simulink model "innerLoopForNav"  (R2024b)
settings: Solver=ode4  StartTime=0.0  StopTime=60  FixedStep=0.02  RelTol=1e-3
undefined symbols (not defined in the file): euler_0, V_0
libraries: simulink x7
settings Model: Creator=yuanjiayi  LastModifiedBy=yuanjiayi

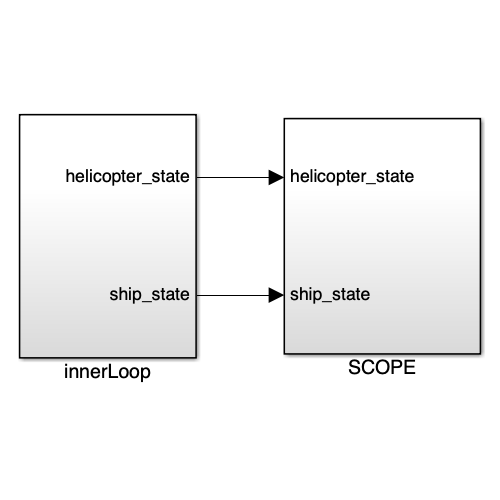
[thumbnail: Simulink's stored preview of the top-level diagram]
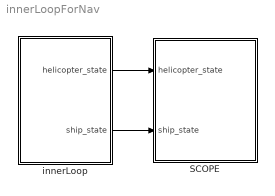
== system innerLoopForNav ==
  SCOPE : Subsystem
  innerLoop : Subsystem
  wires:
  innerLoop/1(helicopter_state) -> SCOPE/1(helicopter_state)
  innerLoop/2(ship_state) -> SCOPE/2(ship_state)

== system innerLoopForNav/SCOPE ==
  helicopter_state : Inport
  ship_state : Inport  Port=2
  Demux1 : Demux  Outputs=12
  Demux2 : Demux  Outputs=12
  Scope : Scope  NumInputPorts=12
  Scope1 : Scope  NumInputPorts=12
  wires:
  Demux2/6 -> Scope1/6  "w"
  Demux2/2 -> Scope1/2  "y"
  helicopter_state/1 -> Demux1/1
  Demux1/1 -> Scope/1  "x"
  Demux1/3 -> Scope/3  "z"
  Demux1/12 -> Scope/12  "r"
  Demux2/9 -> Scope1/9  "psi"
  Demux1/9 -> Scope/9  "psi"
  Demux2/5 -> Scope1/5  "v"
  Demux1/7 -> Scope/7  "phi"
  Demux1/11 -> Scope/11  "q"
  Demux2/4 -> Scope1/4  "u"
  Demux1/2 -> Scope/2  "y"
  Demux1/8 -> Scope/8  "theta"
  Demux1/5 -> Scope/5  "v"
  Demux2/11 -> Scope1/11  "q"
  Demux2/12 -> Scope1/12  "r"
  ship_state/1 -> Demux2/1
  Demux2/3 -> Scope1/3  "z"
  Demux1/10 -> Scope/10  "p"
  Demux2/10 -> Scope1/10  "p"
  Demux2/1 -> Scope1/1  "x"
  Demux2/7 -> Scope1/7  "phi"
  Demux1/4 -> Scope/4  "u"
  Demux2/8 -> Scope1/8  "theta"
  Demux1/6 -> Scope/6  "w"

== system innerLoopForNav/innerLoop ==
  HELI_CONT : Subsystem
  LAND_CMD : Subsystem
  Mux : Mux  Inputs=2
  Plus : Sum
  mps2knots : Gain  Gain=[1/0.514444;1/0.514444;1/0.514444;1;1;1;1;1;1]
  mps2knots1 : Gain  Gain=[1;1;1;1/0.514444;1/0.514444;1/0.514444;1;1;1;1;1;1]
  relistedStates : Selector  InputPortWidth=9  IndexOptions=Index vector (dialog)  Indices=[1 5 2 8 4 9 6 3 7]  OutputSizes=1
  trim_9states : Constant  Value=[V_0; euler_0;zeros(3,1)]
  helicopter_state : Outport
  ship_state : Outport  Port=2
  wires:
  LAND_CMD/1(ref /knots) -> HELI_CONT/1(ref_ned)  "ref_ned / knots"
  LAND_CMD/3(xyz_heli) -> Mux/1
  Mux/1 -> helicopter_state/1
  HELI_CONT/1(V_ned) -> LAND_CMD/1(V_ned / knots)  "V_ned / knots"
  HELI_CONT/2(9states_heli) -> relistedStates/1
  LAND_CMD/2(ship_state) -> mps2knots1/1
  relistedStates/1 -> Plus/1
  Plus/1 -> mps2knots/1
  trim_9states/1 -> Plus/2
  mps2knots/1 -> Mux/2
  mps2knots1/1 -> ship_state/1

== system innerLoopForNav/innerLoop/HELI_CONT ==
  ref_ned : Inport
  SCOPE : Subsystem
  Some methods : Subsystem  Commented=on
  UWV_CONT : Subsystem
  nedToUwv : Subsystem
  V_ned : Outport
  9states_heli : Outport  Port=2
  wires:
  ref_ned/1 -> [ref_ned], nedToUwv/1(In1)
  UWV_CONT/2(euler) -> [euler]
  UWV_CONT/1(V_ned) -> V_ned/1, [V_ned]
  [euler] -> nedToUwv/2(In2)  "eluer / rad"
  nedToUwv/1(ref) -> UWV_CONT/1(ref)  "ref_u,w,v"
  [ref_ned] -> SCOPE/1(ref_ned)
  [V_ned] -> SCOPE/2(V_ned)
  UWV_CONT/3(9states_heli) -> 9states_heli/1

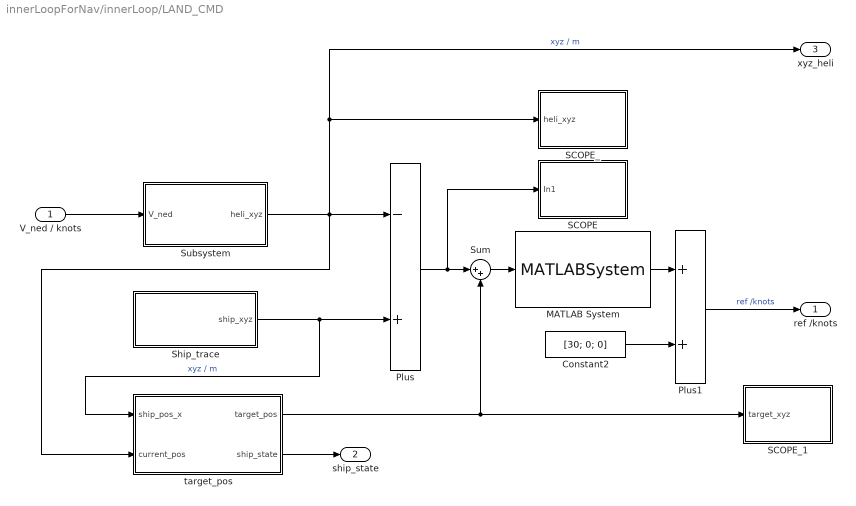
== system innerLoopForNav/innerLoop/LAND_CMD ==
  V_ned / knots : Inport
  Constant2 : Constant  Value=[30; 0; 0]
  MATLAB System : MATLABSystem  System=uvw_Gen  maxDeltaVel_n=1.5  maxDeltaVel_e=0.5  maxDeltaVel_d=1.5  SimulateUsing=Code generation
      mask Type: uvw_Gen
      mask Display:
      | disp('uvw_Gen');
      | port_label('input',1,'Delta_r');
      | port_label('output',1,'Delta_v');
  Plus : Sum  Inputs=-+
  Plus1 : Sum
  "SCOPE " : Subsystem
  SCOPE_ : Subsystem
  SCOPE_1 : Subsystem
  Ship_trace : Subsystem
  Subsystem : Subsystem
  Sum : Sum  Inputs=|++
  target_pos : Subsystem
  ref /knots : Outport
  ship_state : Outport  Port=2
  xyz_heli : Outport  Port=3
  wires:
  Constant2/1 -> Plus1/2
  Plus1/1 -> ref /knots/1  "ref /knots"
  V_ned / knots/1 -> Subsystem/1(V_ned)
  MATLAB System/1 -> Plus1/1
  Subsystem/1(heli_xyz) -> Plus/1, SCOPE_/1(heli_xyz), xyz_heli/1, target_pos/2(current_pos)  "xyz / m"
  Plus/1 -> "SCOPE "/1(In1), Sum/1
  Ship_trace/1(ship_xyz) -> Plus/2, target_pos/1(ship_pos_x)  "xyz / m"
  target_pos/1(target_pos) -> Sum/2, SCOPE_1/1(target_xyz)
  target_pos/2(ship_state) -> ship_state/1
  Sum/1 -> MATLAB System/1

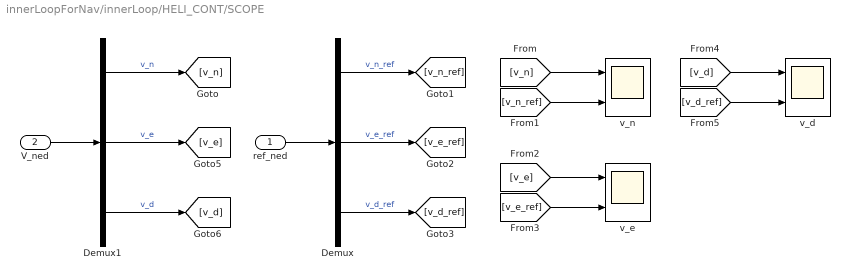
== system innerLoopForNav/innerLoop/HELI_CONT/SCOPE ==
  ref_ned : Inport
  V_ned : Inport  Port=2
  Demux : Demux  Outputs=3
  Demux1 : Demux  Outputs=3
  v_d : Scope  NumInputPorts=2
  v_e : Scope  NumInputPorts=2
  v_n : Scope  NumInputPorts=2
  wires:
  ref_ned/1 -> Demux/1
  V_ned/1 -> Demux1/1
  Demux1/1 -> [v_n]  "v_n"
  Demux/1 -> [v_n_ref]  "v_n_ref"
  [v_n] -> v_n/1
  [v_n_ref] -> v_n/2
  Demux/2 -> [v_e_ref]  "v_e_ref"
  Demux/3 -> [v_d_ref]  "v_d_ref"
  Demux1/2 -> [v_e]  "v_e"
  Demux1/3 -> [v_d]  "v_d"
  [v_e] -> v_e/1
  [v_e_ref] -> v_e/2
  [v_d] -> v_d/1
  [v_d_ref] -> v_d/2

== system innerLoopForNav/innerLoop/HELI_CONT/Some methods ==
  NDI_ : Subsystem  Commented=on
  PID_ : Subsystem  Commented=on
  reference signal : Subsystem  Commented=on

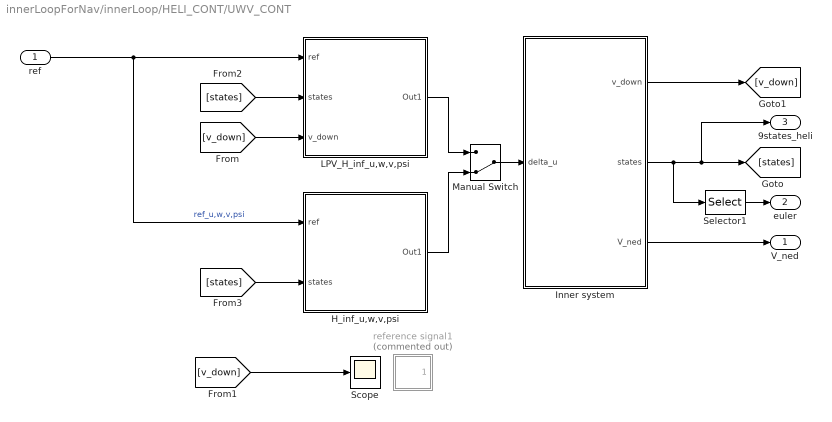
== system innerLoopForNav/innerLoop/HELI_CONT/UWV_CONT ==
  ref : Inport
  H_inf_u,w,v,psi : Subsystem
  Inner system : Subsystem
  LPV_H_inf_u,w,v,psi : Subsystem
  Manual Switch : ManualSwitch  CurrentSetting=0
  Scope : Scope
  Selector1 : Selector  InputPortWidth=9  IndexOptions=Index vector (dialog)  Indices=[8 4 9]  OutputSizes=1
  reference signal1 : Subsystem  Commented=on
  V_ned : Outport
  euler : Outport  Port=2
  9states_heli : Outport  Port=3
  wires:
  Inner system/1(v_down) -> [v_down]
  Inner system/2(states) -> 9states_heli/1, [states], Selector1/1
  Inner system/3(V_ned) -> V_ned/1
  ref/1 -> H_inf_u,w,v,psi/1(ref), LPV_H_inf_u,w,v,psi/1(ref)  "ref_u,w,v,psi"
  [states] -> LPV_H_inf_u,w,v,psi/2(states)
  [v_down] -> LPV_H_inf_u,w,v,psi/3(v_down)
  [v_down] -> Scope/1
  Selector1/1 -> euler/1
  LPV_H_inf_u,w,v,psi/1(Out1) -> Manual Switch/1
  Manual Switch/1 -> Inner system/1(delta_u)
  H_inf_u,w,v,psi/1(Out1) -> Manual Switch/2
  [states] -> H_inf_u,w,v,psi/2(states)

== system innerLoopForNav/innerLoop/HELI_CONT/nedToUwv ==
  In1 : Inport
  In2 : Inport  Port=2
  Constant : Constant  Value=0
  Constant2 : Constant  Value=[V_0]
  Demux2 : Demux  Outputs=3
  Gain : Gain  Gain=0.514444
  MATLAB System : MATLABSystem  System=nedVelToBody  SimulateUsing=Code generation
      mask Type: nedVelToBody
      mask Display:
      | disp('nedVelToBody');
      | port_label('input',1,'V_ned');
      | port_label('input',2,'Euler');
      | port_label('output',1,'V_body');
  Mux : Mux  Inputs=2
  Plus : Sum  Inputs=+-
  Scope3 : Scope  NumInputPorts=3
  Selector : Selector  InputPortWidth=3  IndexOptions=Index vector (dialog)  Indices=[1 3 2]  OutputSizes=1
  filter_phi,theta,psi : Subsystem
  filter_u,w,v,psi : Subsystem  Commented=on
  ref : Outport
  wires:
  filter_phi,theta,psi/1(Out1) -> MATLAB System/2
  Demux2/2 -> Scope3/2  "v"
  Demux2/3 -> Scope3/3  "w"
  In2/1 -> filter_phi,theta,psi/1(In1)
  MATLAB System/1 -> Plus/1, Demux2/1  "V_body_ref"
  Constant/1 -> Mux/2
  In1/1 -> Gain/1
  Demux2/1 -> Scope3/1  "u"
  Plus/1 -> Selector/1
  Constant2/1 -> Plus/2  "V_body_trim"
  Selector/1 -> Mux/1
  Gain/1 -> MATLAB System/1
  Mux/1 -> ref/1

== system innerLoopForNav/innerLoop/LAND_CMD/SCOPE  ==
  In1 : Inport
  Demux : Demux  Outputs=3
  Scope : Scope  NumInputPorts=3
  wires:
  Demux/3 -> Scope/3  "delta_z"
  In1/1 -> Demux/1
  Demux/2 -> Scope/2  "delta_y"
  Demux/1 -> Scope/1  "delta_x"

== system innerLoopForNav/innerLoop/LAND_CMD/SCOPE_ ==
  heli_xyz : Inport
  Demux : Demux  Outputs=3
  Gain : Gain  Gain=-1
  MATLAB Function : MATLAB Function  TreatAsAtomicUnit=on
  Scope : Scope  NumInputPorts=3
  Stop Simulation : Stop
  To Workspace : ToWorkspace  VariableName=heli_trace  SampleTime=-1
  wires:
  Demux/3 -> Gain/1  "z"
  heli_xyz/1 -> To Workspace/1, Demux/1
  Demux/2 -> Scope/2  "y"
  Demux/1 -> Scope/1  "x"
  Gain/1 -> MATLAB Function/1(z), Scope/3  "z"
  MATLAB Function/1(shallStop) -> Stop Simulation/1

== system innerLoopForNav/innerLoop/LAND_CMD/SCOPE_1 ==
  target_xyz : Inport
  Demux : Demux  Outputs=3
  Gain : Gain  Gain=-1
  Scope : Scope  NumInputPorts=3
  wires:
  Demux/3 -> Gain/1  "z"
  target_xyz/1 -> Demux/1
  Demux/2 -> Scope/2  "y"
  Demux/1 -> Scope/1  "x"
  Gain/1 -> Scope/3

== system innerLoopForNav/innerLoop/LAND_CMD/Ship_trace ==
  Constant2 : Constant  Value=[30; 0; 0]
  Gain1 : Gain  Gain=0.514444
  Integrator1 : Integrator  InitialCondition=[95;0;0]
  ship_xyz : Outport
  wires:
  Gain1/1 -> Integrator1/1
  Integrator1/1 -> ship_xyz/1
  Constant2/1 -> Gain1/1

== system innerLoopForNav/innerLoop/LAND_CMD/Subsystem ==
  V_ned : Inport
  Gain : Gain  Gain=0.514444
  Integrator : Integrator  InitialCondition=[0;0;-50]
  heli_xyz : Outport
  wires:
  Integrator/1 -> heli_xyz/1
  V_ned/1 -> Gain/1
  Gain/1 -> Integrator/1

== system innerLoopForNav/innerLoop/LAND_CMD/target_pos ==
  ship_pos_x : Inport
  current_pos : Inport  Port=2
  Chart : Stateflow chart  TreatAsAtomicUnit=on
  PredictModel : Subsystem
  Scope : Scope
  Selector : Selector  InputPortWidth=3  IndexOptions=Index vector (dialog)  Indices=[3]  OutputSizes=1
  Selector1 : Selector  InputPortWidth=3  IndexOptions=Index vector (dialog)  Indices=[1]  OutputSizes=1
  Selector2 : Selector  InputPortWidth=3  IndexOptions=Index vector (dialog)  Indices=[1]  OutputSizes=1
  Ship_motion : Subsystem
  To Workspace : ToWorkspace  VariableName=process_state  SampleTime=-1
  vel_cmd : Constant  Value=[30 ;0;0]
  target_pos : Outport
  ship_state : Outport  Port=2
  wires:
  vel_cmd/1 -> Ship_motion/1(In2), PredictModel/1(In2)
  current_pos/1 -> Selector/1, Selector1/1
  Selector/1 -> Chart/2(z)
  PredictModel/1(EI) -> Chart/1(EI)
  Chart/1(target_pos) -> target_pos/1
  Chart/2(state) -> To Workspace/1, Scope/1
  Ship_motion/1(ship_state) -> ship_state/1
  Selector1/1 -> Chart/3(x)
  ship_pos_x/1 -> Selector2/1
  Selector2/1 -> Chart/4(ship_pos_x)

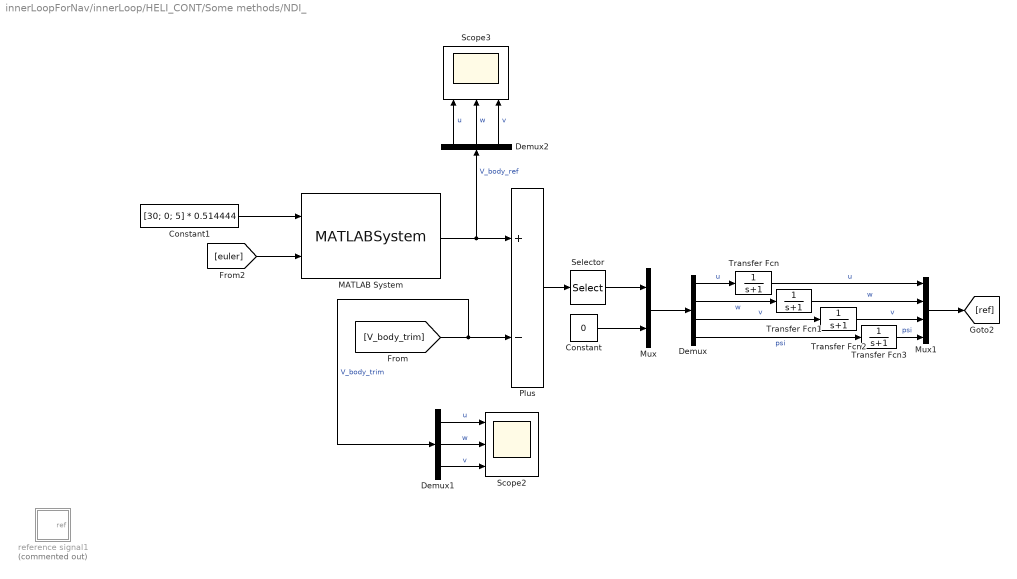
== system innerLoopForNav/innerLoop/HELI_CONT/Some methods/NDI_ ==
  Constant : Constant  Value=0
  Constant1 : Constant  Value=[30; 0; 5] * 0.514444
  Demux : Demux
  Demux1 : Demux  Outputs=3
  Demux2 : Demux  Outputs=3
  MATLAB System : MATLABSystem  System=nedVelToBody  SimulateUsing=Code generation
      mask Type: nedVelToBody
      mask Display:
      | disp('nedVelToBody');
      | port_label('input',1,'V_ned');
      | port_label('input',2,'Euler');
      | port_label('output',1,'V_body');
  Mux : Mux  Inputs=2
  Mux1 : Mux
  Plus : Sum  Inputs=+-
  Scope2 : Scope  NumInputPorts=3
  Scope3 : Scope  NumInputPorts=3
  Selector : Selector  InputPortWidth=3  IndexOptions=Index vector (dialog)  Indices=[1 3 2]  OutputSizes=1
  Transfer Fcn{,1..3} (4 alike) : TransferFcn  Denominator=[1 1]
  reference signal1 : Subsystem  Commented=on
  wires:
  Demux/3 -> Transfer Fcn2/1  "v"
  Demux2/2 -> Scope3/2  "w"
  Demux1/1 -> Scope2/1  "u"
  Mux/1 -> Demux/1
  MATLAB System/1 -> Plus/1, Demux2/1  "V_body_ref"
  Transfer Fcn3/1 -> Mux1/4  "psi"
  Demux2/3 -> Scope3/3  "v"
  Demux1/2 -> Scope2/2  "w"
  Constant1/1 -> MATLAB System/1
  Demux/1 -> Transfer Fcn/1  "u"
  Plus/1 -> Selector/1
  Mux1/1 -> [ref]
  Transfer Fcn1/1 -> Mux1/2  "w"
  Selector/1 -> Mux/1
  [euler] -> MATLAB System/2
  Demux/2 -> Transfer Fcn1/1  "w"
  Transfer Fcn/1 -> Mux1/1  "u"
  [V_body_trim] -> Demux1/1, Plus/2  "V_body_trim"
  Demux/4 -> Transfer Fcn3/1  "psi"
  Transfer Fcn2/1 -> Mux1/3  "v"
  Demux2/1 -> Scope3/1  "u"
  Demux1/3 -> Scope2/3  "v"
  Constant/1 -> Mux/2

== system innerLoopForNav/innerLoop/HELI_CONT/Some methods/PID_ ==
  Gain : Gain  Gain=0.514444
  Mux : Mux  Inputs=3
  Mux1 : Mux  Inputs=2
  Plus : Sum  Inputs=+-
  Scope1 : Scope
  filter & selector : Subsystem
  psi_ref : Constant  Value=0
  v_d_ref / knots : Constant  Value=5.0
  v_e_ref / knots : Constant  Value=0
  v_n_ref / knots : Constant  Value=30
  Out1 : Outport
  wires:
  Mux1/1 -> Out1/1
  v_d_ref / knots/1 -> Mux/3
  psi_ref/1 -> Mux1/2
  filter & selector/1(Out1) -> Scope1/1, Gain/1
  Gain/1 -> Mux1/1
  [ned] -> Plus/2
  Mux/1 -> Plus/1
  v_n_ref / knots/1 -> Mux/1
  Plus/1 -> filter & selector/1(In1)
  v_e_ref / knots/1 -> Mux/2

== system innerLoopForNav/innerLoop/HELI_CONT/Some methods/reference signal ==
  Constant : Constant  Value=0.5
  Mux : Mux
  Sine Wave : Sin  Amplitude=0.0  Frequency=0.2  SampleTime=0
  Sine Wave2 : Sin  Amplitude=0.0  Frequency=0.15  Phase=pi / 4  SampleTime=0
  Sine Wave3 : Sin  Amplitude=0.0  Frequency=0.15  Phase=pi / 4  SampleTime=0
  Out1 : Outport
  wires:
  Sine Wave/1 -> Mux/1  "ref_delta_u"
  Mux/1 -> Out1/1
  Constant/1 -> Mux/2  "ref_delta_w"
  Sine Wave2/1 -> Mux/3  "ref_delta_v"
  Sine Wave3/1 -> Mux/4  "ref_delta_psi"

== system innerLoopForNav/innerLoop/HELI_CONT/UWV_CONT/H_inf_u,w,v,psi ==
  ref : Inport
  states : Inport  Port=2
  MATLAB System : MATLABSystem  System=H_inf  PlantA=A_0  PlantB=B_0  ControlledStateIndices=[ 1, 2, 5, 9]  SampleTime=0.02  DKIterations=10  SelectedIteration=6  FrequencyGrid=logspace( -3, 3, 300 )  DiscretizationMethod=tustin  PerformanceA=0.005  PerformanceM=2  PerformanceBandwidth=1  UncertaintyZero=0.2  UncertaintyDenS=0.5  UncertaintyDen0=1  EnableInputSaturation=false  InputLowerLimit=-0.01 * ones( 4, 1 )  InputUpperLimit=0.01 * ones( 4, 1 )  SimulateUsing=Interpreted execution
      mask Type: H_inf
      mask Display:
      | disp('H_inf');
      | port_label('input',1,'r');
      | port_label('input',2,'y');
      | port_label('output',1,'delta');
  SCOPE : Subsystem
  Selector2 : Selector  InputPortWidth=9  IndexOptions=Index vector (dialog)  Indices=[1 2 5 9]  OutputSizes=1
  Out1 : Outport
  wires:
  states/1 -> Selector2/1
  Selector2/1 -> MATLAB System/2, SCOPE/2(y)  "u,w,v,psi"
  MATLAB System/1 -> Out1/1
  ref/1 -> MATLAB System/1, SCOPE/1(ref)

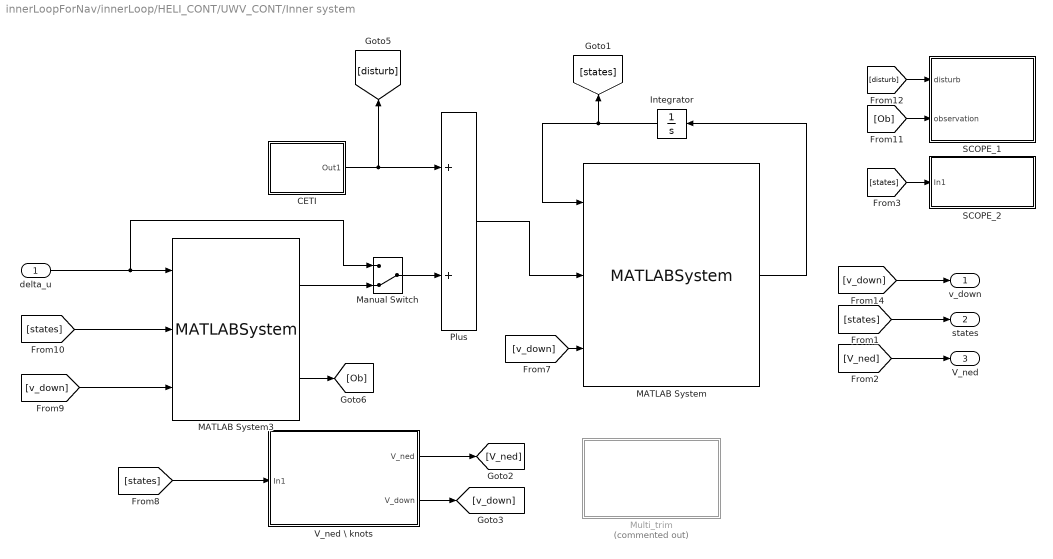
== system innerLoopForNav/innerLoop/HELI_CONT/UWV_CONT/Inner system ==
  delta_u : Inport
  CETI : Subsystem
  Integrator : Integrator  InitialCondition=[0.0;0.0;0.0;0.0;0.0;0.0;0.0;0.0;0.0]
  MATLAB System : MATLABSystem  System=multi_lin_sys  A_10=A_10  B_10=B_10  A_5=A_5  B_5=B_5  A_0=A_0  B_0=B_0  ClampSchedulingVariable=true  SimulateUsing=Interpreted execution
      mask Type: multi_lin_sys
      mask Display:
      | disp('multi_lin_sys');
      | port_label('input',1,'x');
      | port_label('input',2,'delta');
      | port_label('input',3,'v_down');
      | port_label('output',1,'x_dot');
  MATLAB System3 : MATLABSystem  System=LPV_NDO  A_10=A_10  B_10=B_10  A_5=A_5  B_5=B_5  A_0=A_0  B_0=B_0  SampleTime=0.02  ObserverBandwidth=50  ObserverGain_10=[]  ObserverGain_5=[]  ObserverGain_0=[]  DisturbanceFilterBandwidth=0  EnableDisturbanceLimit=true  DisturbanceLowerLimit=[ -0.05; -0.05; -0.05; -0.05 ]  DisturbanceUpperLimit=[ 0.05; 0.05; 0.05; 0.05 ]  EnableInputSaturation=false  InputLowerLimit=[ -inf; -inf; -inf; -inf ]  InputUpperLimit=[ inf; inf; inf; inf ]  ClampSchedulingVariable=true  SimulateUsing=Code generation
      mask Type: LPV_NDO
      mask Display:
      | disp('LPV_NDO');
      | port_label('input',1,'u0');
      | port_label('input',2,'x');
      | port_label('input',3,'v_down');
      | port_label('output',1,'u_comp');
      | port_label('output',2,'d_hat');
  Manual Switch : ManualSwitch  CurrentSetting=0
  Multi_trim : Subsystem  Commented=on
  Plus : Sum
  SCOPE_1 : Subsystem
  SCOPE_2 : Subsystem
  V_ned \ knots : Subsystem
  v_down : Outport
  states : Outport  Port=2
  V_ned : Outport  Port=3
  wires:
  [states] -> V_ned \ knots/1(In1)
  [v_down] -> MATLAB System/3
  [states] -> MATLAB System3/2
  MATLAB System/1 -> Integrator/1
  Integrator/1 -> MATLAB System/1, [states]
  CETI/1(Out1) -> Plus/1, [disturb]
  MATLAB System3/2 -> [Ob]
  [v_down] -> MATLAB System3/3
  delta_u/1 -> Manual Switch/1, MATLAB System3/1
  [v_down] -> v_down/1
  [Ob] -> SCOPE_1/2(observation)
  [disturb] -> SCOPE_1/1(disturb)
  [states] -> states/1
  V_ned \ knots/1("V_ned ") -> [V_ned]
  V_ned \ knots/2(V_down) -> [v_down]
  [V_ned] -> V_ned/1
  [states] -> SCOPE_2/1(In1)
  Plus/1 -> MATLAB System/2
  Manual Switch/1 -> Plus/2
  MATLAB System3/1 -> Manual Switch/2

== system innerLoopForNav/innerLoop/HELI_CONT/UWV_CONT/LPV_H_inf_u,w,v,psi ==
  ref : Inport
  states : Inport  Port=2
  v_down : Inport  Port=3
  CONT_u,w,v,psi : MATLABSystem  System=LPV_H_inf  A_10=A_10  B_10=B_10  A_5=A_5  B_5=B_5  A_0=A_0  B_0=B_0  ControlledStateIndices=[ 1, 2, 5, 9]  SampleTime=0.02  DKIterations=10  SelectedIteration=6  FrequencyGrid=logspace( -3, 3, 300 )  DiscretizationMethod=tustin  PerformanceA=0.005  PerformanceM=2  PerformanceBandwidth=1  UncertaintyZero=0.2  UncertaintyDenS=0.5  UncertaintyDen0=1  ClampSchedulingVariable=true  EnableInputSaturation=false  InputLowerLimit=-0.01 * ones( 4, 1 )  InputUpperLimit=0.01 * ones( 4, 1 )  SimulateUsing=Interpreted execution
      mask Type: LPV_H_inf
      mask Display:
      | disp('LPV_H_inf');
      | port_label('input',1,'r');
      | port_label('input',2,'y');
      | port_label('input',3,'v_down');
      | port_label('output',1,'delta');
  SCOPE : Subsystem
  Selector2 : Selector  InputPortWidth=9  IndexOptions=Index vector (dialog)  Indices=[1 2 5 9]  OutputSizes=1
  Out1 : Outport
  wires:
  states/1 -> Selector2/1
  Selector2/1 -> SCOPE/2(y), CONT_u,w,v,psi/2  "u,w,v,psi"
  v_down/1 -> CONT_u,w,v,psi/3  "v_down / knots"
  CONT_u,w,v,psi/1 -> Out1/1
  ref/1 -> SCOPE/1(ref), CONT_u,w,v,psi/1

== system innerLoopForNav/innerLoop/HELI_CONT/UWV_CONT/reference signal1 ==
  Mux : Mux
  Sine Wave : Sin  Amplitude=0.1  Frequency=0.2  SampleTime=0
  Sine Wave1 : Sin  Amplitude=0.1  Frequency=0.15  Phase=pi / 4  SampleTime=0
  Sine Wave2 : Sin  Amplitude=0.1  Frequency=0.15  Phase=pi / 4  SampleTime=0
  Sine Wave3 : Sin  Amplitude=0.0  Frequency=0.15  Phase=pi / 4  SampleTime=0
  Out1 : Outport
  wires:
  Sine Wave/1 -> Mux/1
  Mux/1 -> Out1/1
  Sine Wave1/1 -> Mux/2
  Sine Wave2/1 -> Mux/3
  Sine Wave3/1 -> Mux/4

== system innerLoopForNav/innerLoop/HELI_CONT/nedToUwv/filter_phi,theta,psi ==
  In1 : Inport
  Demux : Demux  Outputs=3
  Mux1 : Mux  Inputs=3
  Transfer Fcn : TransferFcn  Denominator=[10 1]
  Transfer Fcn1 : TransferFcn  Denominator=[10 1]
  Transfer Fcn2 : TransferFcn  Denominator=[10 1]
  Out1 : Outport
  wires:
  Mux1/1 -> Out1/1
  Demux/2 -> Transfer Fcn1/1  "theta"
  Demux/3 -> Transfer Fcn2/1  "psi"
  In1/1 -> Demux/1
  Transfer Fcn1/1 -> Mux1/2  "theta"
  Demux/1 -> Transfer Fcn/1  "phi"
  Transfer Fcn2/1 -> Mux1/3  "psi"
  Transfer Fcn/1 -> Mux1/1  "phi"

== system innerLoopForNav/innerLoop/HELI_CONT/nedToUwv/filter_u,w,v,psi ==
  In1 : Inport
  Demux : Demux
  Mux1 : Mux
  Transfer Fcn{,1..3} (4 alike) : TransferFcn  Denominator=[1 1]
  Out1 : Outport
  wires:
  Mux1/1 -> Out1/1
  Demux/2 -> Transfer Fcn1/1  "w"
  Transfer Fcn3/1 -> Mux1/4  "psi"
  Demux/4 -> Transfer Fcn3/1  "psi"
  Demux/3 -> Transfer Fcn2/1  "v"
  In1/1 -> Demux/1
  Transfer Fcn1/1 -> Mux1/2  "w"
  Demux/1 -> Transfer Fcn/1  "u"
  Transfer Fcn2/1 -> Mux1/3  "v"
  Transfer Fcn/1 -> Mux1/1  "u"

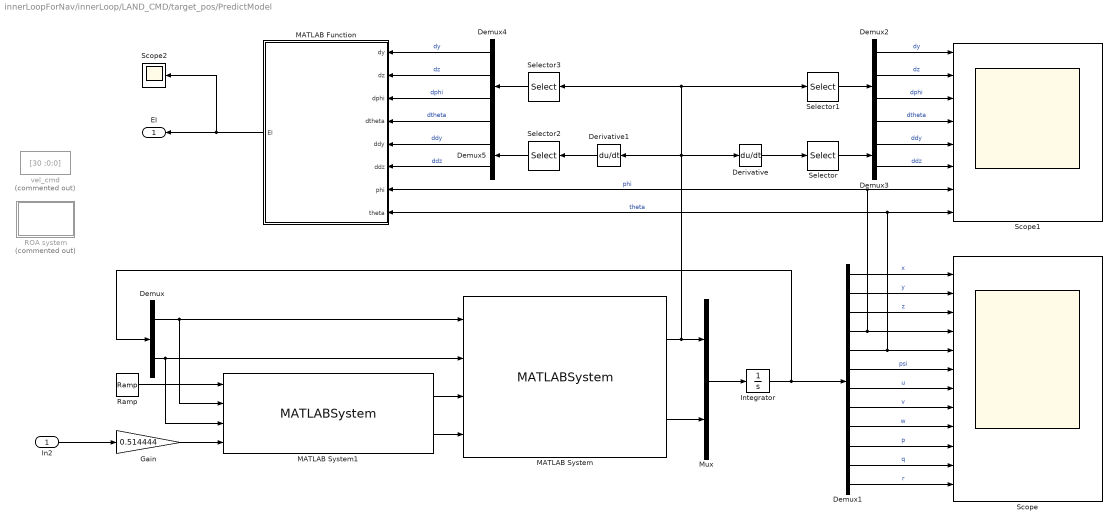
== system innerLoopForNav/innerLoop/LAND_CMD/target_pos/PredictModel ==
  In2 : Inport
  Demux : Demux  Outputs=2
  Demux1 : Demux  Outputs=12
  Demux2 : Demux
  Demux3 : Demux  Outputs=2
  Demux4 : Demux
  Demux5 : Demux  Outputs=2
  Derivative : Derivative
  Derivative1 : Derivative
  Gain : Gain  Gain=0.514444
  Integrator : Integrator  InitialCondition=[95;0;0;0;0;0;30 * 0.51444;0;0;0;0;0]
  MATLAB Function : MATLAB Function  TreatAsAtomicUnit=on
  MATLAB System : MATLABSystem  System=ship_motion_model_2  MassMatrix=MassMatrix  AddedMass=AddedMass  LinearDamping=LinearDamping  QuadraticDamping=zeros( 6 )  RestoringMatrix=RestoringMatrix  RestoringEquilibrium=zeros( 6, 1 )  EulerCosineTolerance=1.0e-8  SimulateUsing=Interpreted execution
      mask Type: ship_motion_model_2
      mask Display:
      | disp(['Ship Motion' char(10) 'Eq. (5)']);
      | port_label('input',1,'eta');
      | port_label('input',2,'nu');
      | port_label('input',3,'tau');
      | port_label('input',4,'F_DI');
      | port_label('output',1,'eta_dot');
      | port_label('output',2,'nu_dot');
  MATLAB System1 : MATLABSystem  System=tauAndFDI  ShipLength=70.2  ShipBeam=11.0  ShipDraught=3.5  DisplacementMass=1.2e6  WaterplaneCoefficient=0.75  TransverseGM=1.5  LongitudinalGM=200  WaterDensity=1025  Gravity=9.80665  DesiredHeading=0  DesiredRollAngle=0  DesiredPitchAngle=0  HeadingCommandSpeedThreshold=0.10  TranslationTimeConstant=[ 3; 4; 2.5 ]  NominalRestoringEquilibrium=zeros( 6, 1 )  ControlNaturalFrequency=[ 0; 0; 0; 0; 0; 0.10 ]  ControlDampingRatio=[ 0; 0; 0; 0; 0; 1.0 ]  WaveFeedforwardGain=[ 0.95; 0.85; 0.50; 0; 0; 0.80 ]  MinimumControlLoad=[ -0.25e6; -0.5e6; -8e6; -1; -1; -15e6 ]  MaximumControlLoad=[ 0.60e6; 0.5e6; 8e6; 1; 1; 15e6 ]  SignificantWaveHeight=2.0  PeakPeriod=11.2  RelativeWaveDirectionDeg=150  MinimumWaveFrequency=0.20  MaximumWaveFrequency=2.00  NumberOfWaveComponents=64  RandomSeed=16  DiffractionScale=1.10  SurgeExcitationCoefficient=0.25  SwayExcitationCoefficient=0.55  HeaveExcitationCoefficient=0.70  RollExcitationCoefficient=1.00  PitchExcitationCoefficient=1.00  YawExcitationCoefficient=0.18  SimulateUsing=Interpreted execution
      mask Type: tauAndFDI
      mask Display:
      | disp(['Control + Wave Loads' char(10) 'NED velocity command']);
      | port_label('input',1,'t');
      | port_label('input',2,'eta');
      | port_label('input',3,'nu');
      | port_label('input',4,'velocity_command_NED');
      | port_label('output',1,'tau');
      | port_label('output',2,'F_DI');
  Mux : Mux  Inputs=2
  ROA system : Subsystem  Commented=on
  Ramp : simulink/Sources/Ramp  slope=1  start=0  InitialOutput=0
  Scope : Scope  NumInputPorts=12
  Scope1 : Scope  NumInputPorts=8
  Scope2 : Scope
  Selector : Selector  InputPortWidth=6  IndexOptions=Index vector (dialog)  Indices=[2 3]  OutputSizes=1
  Selector1 : Selector  InputPortWidth=6  IndexOptions=Index vector (dialog)  Indices=[2 3 4 5]  OutputSizes=1
  Selector2 : Selector  InputPortWidth=6  IndexOptions=Index vector (dialog)  Indices=[2 3]  OutputSizes=1
  Selector3 : Selector  InputPortWidth=6  IndexOptions=Index vector (dialog)  Indices=[2 3 4 5]  OutputSizes=1
  vel_cmd : Constant  Commented=on  Value=[30 ;0;0]
  EI : Outport
  wires:
  Demux4/3 -> MATLAB Function/3(dphi)  "dphi"
  Demux2/1 -> Scope1/1  "dy"
  Demux2/3 -> Scope1/3  "dphi"
  In2/1 -> Gain/1
  Selector3/1 -> Demux4/1
  Demux5/1 -> MATLAB Function/5(ddy)  "ddy"
  Demux4/1 -> MATLAB Function/1(dy)  "dy"
  Demux2/2 -> Scope1/2  "dz"
  Gain/1 -> MATLAB System1/4
  Selector1/1 -> Demux2/1
  Selector/1 -> Demux3/1
  Demux1/6 -> Scope/6  "psi"
  Demux4/4 -> MATLAB Function/4(dtheta)  "dtheta"
  Demux4/2 -> MATLAB Function/2(dz)  "dz"
  Demux/1 -> MATLAB System1/2, MATLAB System/1
  Demux5/2 -> MATLAB Function/6(ddz)  "ddz"
  Integrator/1 -> Demux/1, Demux1/1
  Demux2/4 -> Scope1/4  "dtheta"
  Demux3/1 -> Scope1/5  "ddy"
  Derivative1/1 -> Selector2/1
  MATLAB System1/2 -> MATLAB System/4
  Demux3/2 -> Scope1/6  "ddz"
  Demux1/5 -> MATLAB Function/8(theta), Scope1/8, Scope/5  "theta"
  Derivative/1 -> Selector/1
  MATLAB System/1 -> Selector3/1, Selector1/1, Derivative1/1, Derivative/1, Mux/1
  Demux1/7 -> Scope/7  "u"
  Demux1/3 -> Scope/3  "z"
  Demux1/11 -> Scope/11  "q"
  Ramp/1 -> MATLAB System1/1
  Demux1/1 -> Scope/1  "x"
  Mux/1 -> Integrator/1
  Demux/2 -> MATLAB System1/3, MATLAB System/2
  Demux1/8 -> Scope/8  "v"
  Demux1/4 -> Scope/4, MATLAB Function/7(phi), Scope1/7  "phi"
  Demux1/2 -> Scope/2  "y"
  Demux1/12 -> Scope/12  "r"
  Demux1/10 -> Scope/10  "p"
  MATLAB System/2 -> Mux/2
  MATLAB System1/1 -> MATLAB System/3
  Demux1/9 -> Scope/9  "w"
  Selector2/1 -> Demux5/1
  MATLAB Function/1(EI) -> Scope2/1, EI/1

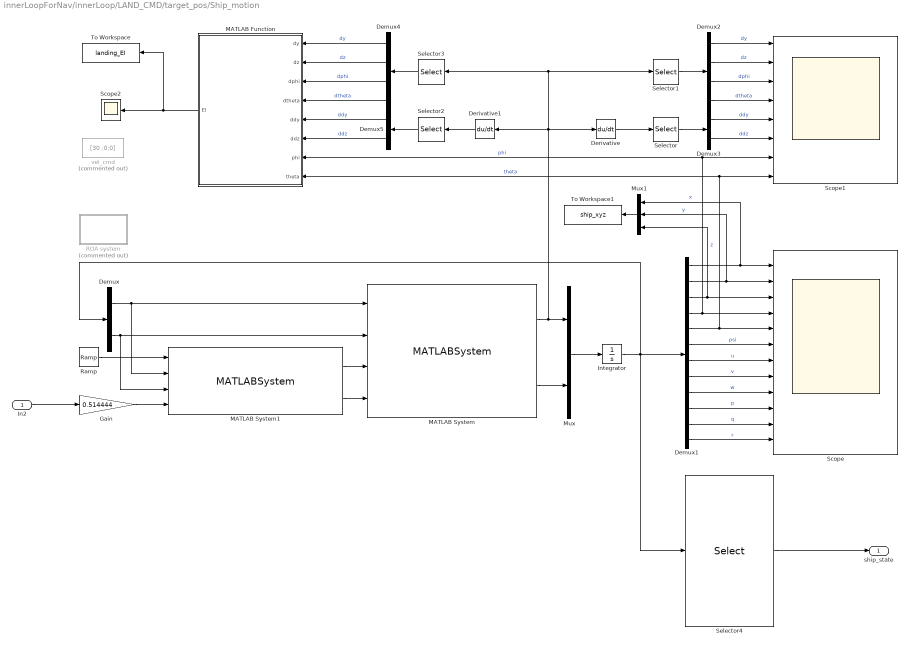
== system innerLoopForNav/innerLoop/LAND_CMD/target_pos/Ship_motion ==
  In2 : Inport
  Demux : Demux  Outputs=2
  Demux1 : Demux  Outputs=12
  Demux2 : Demux
  Demux3 : Demux  Outputs=2
  Demux4 : Demux
  Demux5 : Demux  Outputs=2
  Derivative : Derivative
  Derivative1 : Derivative
  Gain : Gain  Gain=0.514444
  Integrator : Integrator  InitialCondition=[95;0;0;0;0;0;30 * 0.51444;0;0;0;0;0]
  MATLAB Function : MATLAB Function  TreatAsAtomicUnit=on
  MATLAB System : MATLABSystem  System=ship_motion_model_2  MassMatrix=MassMatrix  AddedMass=AddedMass  LinearDamping=LinearDamping  QuadraticDamping=zeros( 6 )  RestoringMatrix=RestoringMatrix  RestoringEquilibrium=zeros( 6, 1 )  EulerCosineTolerance=1.0e-8  SimulateUsing=Interpreted execution
      mask Type: ship_motion_model_2
      mask Display:
      | disp(['Ship Motion' char(10) 'Eq. (5)']);
      | port_label('input',1,'eta');
      | port_label('input',2,'nu');
      | port_label('input',3,'tau');
      | port_label('input',4,'F_DI');
      | port_label('output',1,'eta_dot');
      | port_label('output',2,'nu_dot');
  MATLAB System1 : MATLABSystem  System=tauAndFDI  ShipLength=70.2  ShipBeam=11.0  ShipDraught=3.5  DisplacementMass=1.2e6  WaterplaneCoefficient=0.75  TransverseGM=1.5  LongitudinalGM=200  WaterDensity=1025  Gravity=9.80665  DesiredHeading=0  DesiredRollAngle=0  DesiredPitchAngle=0  HeadingCommandSpeedThreshold=0.10  TranslationTimeConstant=[ 3; 4; 2.5 ]  NominalRestoringEquilibrium=zeros( 6, 1 )  ControlNaturalFrequency=[ 0; 0; 0; 0; 0; 0.10 ]  ControlDampingRatio=[ 0; 0; 0; 0; 0; 1.0 ]  WaveFeedforwardGain=[ 0.95; 0.85; 0.50; 0; 0; 0.80 ]  MinimumControlLoad=[ -0.25e6; -0.5e6; -8e6; -1; -1; -15e6 ]  MaximumControlLoad=[ 0.60e6; 0.5e6; 8e6; 1; 1; 15e6 ]  SignificantWaveHeight=2.0  PeakPeriod=11.2  RelativeWaveDirectionDeg=150  MinimumWaveFrequency=0.20  MaximumWaveFrequency=2.00  NumberOfWaveComponents=64  RandomSeed=16  DiffractionScale=1.10  SurgeExcitationCoefficient=0.25  SwayExcitationCoefficient=0.55  HeaveExcitationCoefficient=0.70  RollExcitationCoefficient=1.00  PitchExcitationCoefficient=1.00  YawExcitationCoefficient=0.18  SimulateUsing=Interpreted execution
      mask Type: tauAndFDI
      mask Display:
      | disp(['Control + Wave Loads' char(10) 'NED velocity command']);
      | port_label('input',1,'t');
      | port_label('input',2,'eta');
      | port_label('input',3,'nu');
      | port_label('input',4,'velocity_command_NED');
      | port_label('output',1,'tau');
      | port_label('output',2,'F_DI');
  Mux : Mux  Inputs=2
  Mux1 : Mux  Inputs=3
  ROA system : Subsystem  Commented=on
  Ramp : simulink/Sources/Ramp  slope=1  start=5  InitialOutput=0
  Scope : Scope  NumInputPorts=12
  Scope1 : Scope  NumInputPorts=8
  Scope2 : Scope
  Selector : Selector  InputPortWidth=6  IndexOptions=Index vector (dialog)  Indices=[2 3]  OutputSizes=1
  Selector1 : Selector  InputPortWidth=6  IndexOptions=Index vector (dialog)  Indices=[2 3 4 5]  OutputSizes=1
  Selector2 : Selector  InputPortWidth=6  IndexOptions=Index vector (dialog)  Indices=[2 3]  OutputSizes=1
  Selector3 : Selector  InputPortWidth=6  IndexOptions=Index vector (dialog)  Indices=[2 3 4 5]  OutputSizes=1
  Selector4 : Selector  InputPortWidth=12  IndexOptions=Index vector (dialog)  Indices=[1 2 3 7 8 9 4 5 6 10 11 12]  OutputSizes=1
  To Workspace : ToWorkspace  VariableName=landing_EI  SampleTime=-1
  To Workspace1 : ToWorkspace  VariableName=ship_xyz  SampleTime=-1
  vel_cmd : Constant  Commented=on  Value=[30 ;0;0]
  ship_state : Outport
  wires:
  Demux2/1 -> Scope1/1  "dy"
  Demux2/3 -> Scope1/3  "dphi"
  In2/1 -> Gain/1
  Demux2/2 -> Scope1/2  "dz"
  Gain/1 -> MATLAB System1/4
  Selector1/1 -> Demux2/1
  Selector/1 -> Demux3/1
  Demux1/6 -> Scope/6  "psi"
  Demux/1 -> MATLAB System1/2, MATLAB System/1
  Integrator/1 -> Demux1/1, Selector4/1, Demux/1
  Demux2/4 -> Scope1/4  "dtheta"
  Demux3/1 -> Scope1/5  "ddy"
  MATLAB System1/2 -> MATLAB System/4
  Demux3/2 -> Scope1/6  "ddz"
  Derivative/1 -> Selector/1
  Demux1/7 -> Scope/7  "u"
  Demux1/3 -> Mux1/3, Scope/3  "z"
  Demux1/11 -> Scope/11  "q"
  Ramp/1 -> MATLAB System1/1
  Demux1/1 -> Mux1/1, Scope/1  "x"
  Mux/1 -> Integrator/1
  Demux/2 -> MATLAB System1/3, MATLAB System/2
  Demux1/8 -> Scope/8  "v"
  Demux1/2 -> Mux1/2, Scope/2  "y"
  Demux1/12 -> Scope/12  "r"
  Demux1/10 -> Scope/10  "p"
  MATLAB System/2 -> Mux/2
  MATLAB System1/1 -> MATLAB System/3
  Demux1/9 -> Scope/9  "w"
  Demux4/4 -> MATLAB Function/4(dtheta)  "dtheta"
  Derivative1/1 -> Selector2/1
  MATLAB Function/1(EI) -> To Workspace/1, Scope2/1
  MATLAB System/1 -> Selector3/1, Selector1/1, Derivative/1, Derivative1/1, Mux/1
  Demux4/2 -> MATLAB Function/2(dz)  "dz"
  Demux5/2 -> MATLAB Function/6(ddz)  "ddz"
  Demux1/5 -> MATLAB Function/8(theta), Scope1/8, Scope/5  "theta"
  Selector3/1 -> Demux4/1
  Selector2/1 -> Demux5/1
  Demux1/4 -> Scope/4, MATLAB Function/7(phi), Scope1/7  "phi"
  Demux4/3 -> MATLAB Function/3(dphi)  "dphi"
  Demux4/1 -> MATLAB Function/1(dy)  "dy"
  Demux5/1 -> MATLAB Function/5(ddy)  "ddy"
  Mux1/1 -> To Workspace1/1
  Selector4/1 -> ship_state/1

== system innerLoopForNav/innerLoop/HELI_CONT/Some methods/NDI_/reference signal1 ==
  Mux : Mux
  Sine Wave : Sin  Amplitude=0  Frequency=0.2  SampleTime=0
  Sine Wave1 : Sin  Amplitude=0  Frequency=0.15  Phase=pi / 4  SampleTime=0
  Sine Wave2 : Sin  Amplitude=0  Frequency=0.15  Phase=pi / 4  SampleTime=0
  Sine Wave3 : Sin  Amplitude=0.0  Frequency=0.15  Phase=pi / 4  SampleTime=0
  ref : Outport
  wires:
  Sine Wave/1 -> Mux/1
  Mux/1 -> ref/1
  Sine Wave1/1 -> Mux/2
  Sine Wave2/1 -> Mux/3
  Sine Wave3/1 -> Mux/4

== system innerLoopForNav/innerLoop/HELI_CONT/Some methods/PID_/filter & selector ==
  In1 : Inport
  Demux : Demux  Outputs=3
  Mux1 : Mux  Inputs=3
  Selector : Selector  InputPortWidth=3  IndexOptions=Index vector (dialog)  Indices=[1 3 2]  OutputSizes=1
  Transfer Fcn : TransferFcn  Denominator=[1 1]
  Transfer Fcn1 : TransferFcn  Denominator=[1 1]
  Transfer Fcn2 : TransferFcn  Denominator=[1 1]
  Out1 : Outport
  wires:
  Mux1/1 -> Selector/1
  Demux/3 -> Transfer Fcn2/1
  Transfer Fcn1/1 -> Mux1/2
  Transfer Fcn2/1 -> Mux1/3
  Demux/1 -> Transfer Fcn/1
  In1/1 -> Demux/1
  Transfer Fcn/1 -> Mux1/1
  Demux/2 -> Transfer Fcn1/1
  Selector/1 -> Out1/1

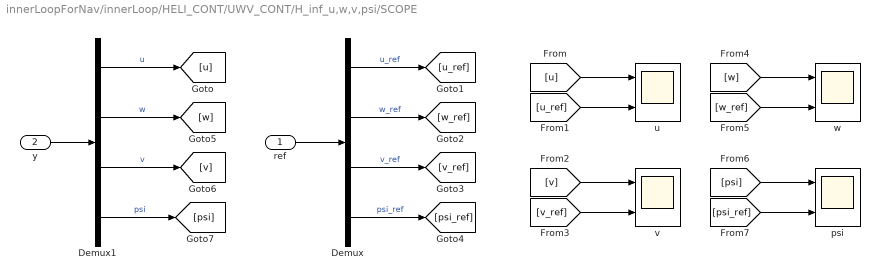
== system innerLoopForNav/innerLoop/HELI_CONT/UWV_CONT/H_inf_u,w,v,psi/SCOPE ==
  ref : Inport
  y : Inport  Port=2
  Demux : Demux
  Demux1 : Demux
  psi : Scope  NumInputPorts=2
  u : Scope  NumInputPorts=2
  v : Scope  NumInputPorts=2
  w : Scope  NumInputPorts=2
  wires:
  ref/1 -> Demux/1
  y/1 -> Demux1/1
  Demux1/1 -> [u]  "u"
  Demux/1 -> [u_ref]  "u_ref"
  [u] -> u/1
  [u_ref] -> u/2
  Demux/2 -> [w_ref]  "w_ref"
  Demux/3 -> [v_ref]  "v_ref"
  Demux/4 -> [psi_ref]  "psi_ref"
  Demux1/2 -> [w]  "w"
  Demux1/3 -> [v]  "v"
  Demux1/4 -> [psi]  "psi"
  [v] -> v/1
  [v_ref] -> v/2
  [w] -> w/1
  [w_ref] -> w/2
  [psi] -> psi/1
  [psi_ref] -> psi/2

== system innerLoopForNav/innerLoop/HELI_CONT/UWV_CONT/Inner system/CETI ==
  Band-Limited White Noise : simulink/Sources/Band-Limited White Noise  Cov=1.0  Ts=0.02  seed=[23341]
  Gain : Gain  Gain=pi / 180
  MATLAB System2 : MATLABSystem  System=CETI  sigma_w=1  Uinf=10  Rm=8.18  Rt=1.68  Ts=0.02  SimulateUsing=Interpreted execution
      mask Type: CETI
      mask Display:
      | disp('CETI');
      | port_label('input',1,'omega_n');
      | port_label('output',1,'du_CETI');
  Out1 : Outport
  wires:
  MATLAB System2/1 -> Gain/1
  Gain/1 -> Out1/1
  Band-Limited White Noise/1 -> MATLAB System2/1

== system innerLoopForNav/innerLoop/HELI_CONT/UWV_CONT/Inner system/Multi_trim ==
  MATLAB System1 : MATLABSystem  System=multi_trim  V_10=V_10  euler_10=euler_10  V_5=V_5  euler_5=euler_5  V_0=V_0  euler_0=euler_0  ClampSchedulingVariable=true  SimulateUsing=Interpreted execution
      mask Type: multi_trim
      mask Display:
      | disp('multi_trim');
      | port_label('input',1,'v_down');
      | port_label('output',1,'trimPos');
  Memory : Memory
  wires:
  MATLAB System1/1 -> [trim]
  [v_down] -> Memory/1
  Memory/1 -> MATLAB System1/1

== system innerLoopForNav/innerLoop/HELI_CONT/UWV_CONT/Inner system/SCOPE_1 ==
  disturb : Inport
  observation : Inport  Port=2
  Demux : Demux
  Demux1 : Demux
  coll : Scope  NumInputPorts=2
  lat : Scope  NumInputPorts=2
  lon : Scope  NumInputPorts=2
  ped : Scope  NumInputPorts=2
  wires:
  disturb/1 -> Demux/1
  observation/1 -> Demux1/1
  Demux/4 -> lat/2  "real"
  Demux1/4 -> lat/1  "ob"
  Demux/3 -> lon/2  "real"
  Demux1/3 -> lon/1  "ob"
  Demux/2 -> coll/2  "real"
  Demux1/2 -> coll/1  "ob"
  Demux/1 -> ped/2  "real"
  Demux1/1 -> ped/1  "ob"

== system innerLoopForNav/innerLoop/HELI_CONT/UWV_CONT/Inner system/SCOPE_2 ==
  In1 : Inport
  Demux : Demux  Outputs=9
  delta_states : Scope  NumInputPorts=9
  wires:
  In1/1 -> Demux/1
  Demux/2 -> delta_states/2  "w"
  Demux/6 -> delta_states/6  "p"
  Demux/3 -> delta_states/3  "q"
  Demux/1 -> delta_states/1  "u"
  Demux/5 -> delta_states/5  "v"
  Demux/7 -> delta_states/7  "r"
  Demux/8 -> delta_states/8  "phi"
  Demux/4 -> delta_states/4  "theta"
  Demux/9 -> delta_states/9  "psi"

== system innerLoopForNav/innerLoop/HELI_CONT/UWV_CONT/Inner system/V_ned \ knots ==
  In1 : Inport
  Constant : Constant  Value=[V_0; euler_0]
  Gain : Gain  Gain=1 / 0.514444
  MATLAB System : MATLABSystem  System=bodyToNedVel  SimulateUsing=Code generation
      mask Type: bodyToNedVel
      mask Display:
      | disp('bodyToNedVel');
      | port_label('input',1,'states');
      | port_label('output',1,'V_ned');
  Plus : Sum
  Selector : Selector  InputPortWidth=9  IndexOptions=Index vector (dialog)  Indices=[1,5,2,8,4,9]  OutputSizes=1
  Selector1 : Selector  InputPortWidth=3  IndexOptions=Index vector (dialog)  Indices=[3]  OutputSizes=1
  Subsystem : Subsystem  Commented=on
  "V_ned " : Outport
  V_down : Outport  Port=2
  wires:
  In1/1 -> Selector/1
  Constant/1 -> Plus/2
  MATLAB System/1 -> Gain/1  "V_ned \\ m/s"
  Selector/1 -> Plus/1  "delta_u,v,w,phi,theta,psi"
  Gain/1 -> Selector1/1, "V_ned "/1  "V_ned \\ knots"
  Plus/1 -> MATLAB System/1
  Selector1/1 -> V_down/1

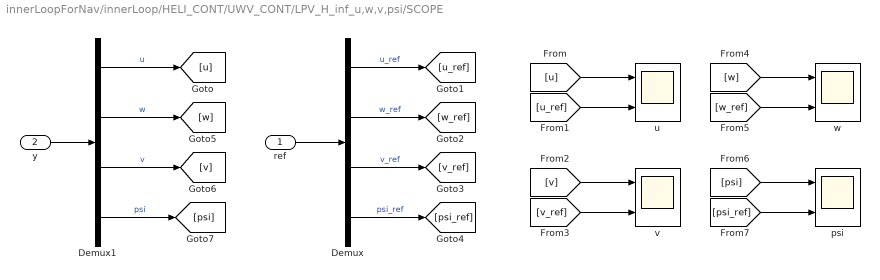
== system innerLoopForNav/innerLoop/HELI_CONT/UWV_CONT/LPV_H_inf_u,w,v,psi/SCOPE ==
  ref : Inport
  y : Inport  Port=2
  Demux : Demux
  Demux1 : Demux
  psi : Scope  NumInputPorts=2
  u : Scope  NumInputPorts=2
  v : Scope  NumInputPorts=2
  w : Scope  NumInputPorts=2
  wires:
  ref/1 -> Demux/1
  y/1 -> Demux1/1
  Demux1/1 -> [u]  "u"
  Demux/1 -> [u_ref]  "u_ref"
  [u] -> u/1
  [u_ref] -> u/2
  Demux/2 -> [w_ref]  "w_ref"
  Demux/3 -> [v_ref]  "v_ref"
  Demux/4 -> [psi_ref]  "psi_ref"
  Demux1/2 -> [w]  "w"
  Demux1/3 -> [v]  "v"
  Demux1/4 -> [psi]  "psi"
  [v] -> v/1
  [v_ref] -> v/2
  [w] -> w/1
  [w_ref] -> w/2
  [psi] -> psi/1
  [psi_ref] -> psi/2

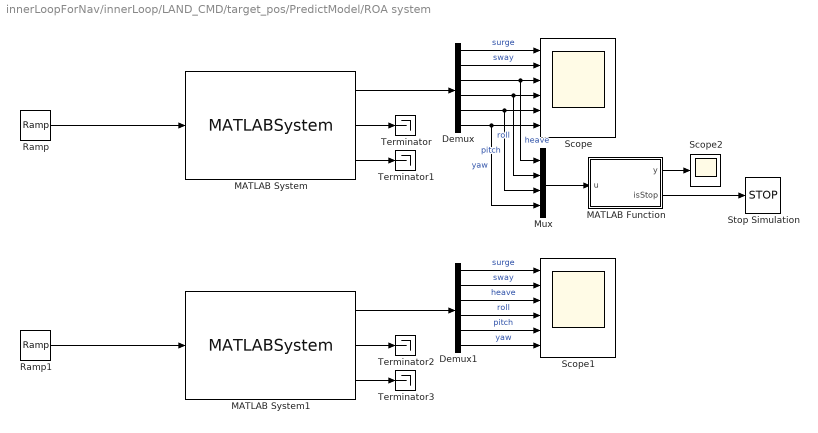
== system innerLoopForNav/innerLoop/LAND_CMD/target_pos/PredictModel/ROA system ==
  Demux : Demux  Outputs=6
  Demux1 : Demux  Outputs=6
  MATLAB Function : MATLAB Function  TreatAsAtomicUnit=on
  MATLAB System : MATLABSystem  System=ship_motion_model  Hs=5.0  g=9.80665  spectrumType=PM  wMin=0.2  wMax=2.5  nComp=48  seed=6  phaseMode=random  RAO=struct()  doWrapAngle=false  SimulateUsing=Interpreted execution
      mask Type: ship_motion_model
      mask Display:
      | disp(['Ship Motion' char(10) '6-DOF']);
      | port_label('input',1,'t');
      | port_label('output',1,'eta');
      | port_label('output',2,'eta_dot');
      | port_label('output',3,'eta_ddot');
  MATLAB System1 : MATLABSystem  System=ship_motion_model  Hs=5.0  g=9.80665  spectrumType=PM  wMin=0.2  wMax=2.5  nComp=48  seed=1  phaseMode=random  RAO=struct()  doWrapAngle=false  SimulateUsing=Interpreted execution
      mask Type: ship_motion_model
      mask Display:
      | disp(['Ship Motion' char(10) '6-DOF']);
      | port_label('input',1,'t');
      | port_label('output',1,'eta');
      | port_label('output',2,'eta_dot');
      | port_label('output',3,'eta_ddot');
  Mux : Mux
  Ramp : simulink/Sources/Ramp  slope=1  start=0  InitialOutput=0
  Ramp1 : simulink/Sources/Ramp  slope=1  start=2.0  InitialOutput=0
  Scope : Scope  NumInputPorts=6
  Scope1 : Scope  NumInputPorts=6
  Scope2 : Scope
  Stop Simulation : Stop
  Terminator{,1..3} (4 alike) : Terminator
  wires:
  MATLAB Function/1(y) -> Scope2/1
  MATLAB Function/2(isStop) -> Stop Simulation/1
  Demux1/1 -> Scope1/1  "surge"
  Demux/1 -> Scope/1  "surge"
  MATLAB System1/3 -> Terminator3/1
  Demux1/6 -> Scope1/6  "yaw"
  MATLAB System/3 -> Terminator1/1
  Demux/3 -> Mux/1, Scope/3  "heave"
  Demux/4 -> Mux/2, Scope/4  "roll"
  Demux/2 -> Scope/2  "sway"
  Ramp1/1 -> MATLAB System1/1
  Demux1/5 -> Scope1/5  "pitch"
  Demux1/2 -> Scope1/2  "sway"
  MATLAB System1/1 -> Demux1/1
  Mux/1 -> MATLAB Function/1(u)
  MATLAB System1/2 -> Terminator2/1
  MATLAB System/1 -> Demux/1
  MATLAB System/2 -> Terminator/1
  Demux/6 -> Mux/4, Scope/6  "yaw"
  Demux/5 -> Mux/3, Scope/5  "pitch"
  Demux1/4 -> Scope1/4  "roll"
  Demux1/3 -> Scope1/3  "heave"
  Ramp/1 -> MATLAB System/1

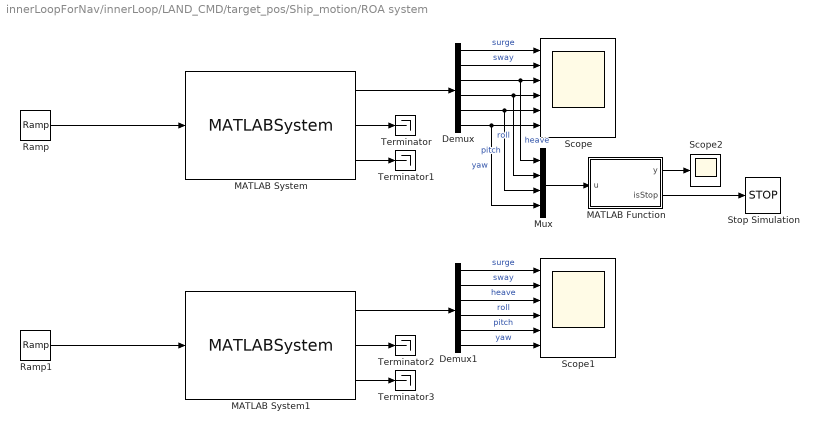
== system innerLoopForNav/innerLoop/LAND_CMD/target_pos/Ship_motion/ROA system ==
  Demux : Demux  Outputs=6
  Demux1 : Demux  Outputs=6
  MATLAB Function : MATLAB Function  TreatAsAtomicUnit=on
  MATLAB System : MATLABSystem  System=ship_motion_model  Hs=5.0  g=9.80665  spectrumType=PM  wMin=0.2  wMax=2.5  nComp=48  seed=6  phaseMode=random  RAO=struct()  doWrapAngle=false  SimulateUsing=Interpreted execution
      mask Type: ship_motion_model
      mask Display:
      | disp(['Ship Motion' char(10) '6-DOF']);
      | port_label('input',1,'t');
      | port_label('output',1,'eta');
      | port_label('output',2,'eta_dot');
      | port_label('output',3,'eta_ddot');
  MATLAB System1 : MATLABSystem  System=ship_motion_model  Hs=5.0  g=9.80665  spectrumType=PM  wMin=0.2  wMax=2.5  nComp=48  seed=1  phaseMode=random  RAO=struct()  doWrapAngle=false  SimulateUsing=Interpreted execution
      mask Type: ship_motion_model
      mask Display:
      | disp(['Ship Motion' char(10) '6-DOF']);
      | port_label('input',1,'t');
      | port_label('output',1,'eta');
      | port_label('output',2,'eta_dot');
      | port_label('output',3,'eta_ddot');
  Mux : Mux
  Ramp : simulink/Sources/Ramp  slope=1  start=0  InitialOutput=0
  Ramp1 : simulink/Sources/Ramp  slope=1  start=2.0  InitialOutput=0
  Scope : Scope  NumInputPorts=6
  Scope1 : Scope  NumInputPorts=6
  Scope2 : Scope
  Stop Simulation : Stop
  Terminator{,1..3} (4 alike) : Terminator
  wires:
  MATLAB Function/1(y) -> Scope2/1
  MATLAB Function/2(isStop) -> Stop Simulation/1
  Demux1/1 -> Scope1/1  "surge"
  Demux/1 -> Scope/1  "surge"
  MATLAB System1/3 -> Terminator3/1
  Demux1/6 -> Scope1/6  "yaw"
  MATLAB System/3 -> Terminator1/1
  Demux/3 -> Mux/1, Scope/3  "heave"
  Demux/4 -> Mux/2, Scope/4  "roll"
  Demux/2 -> Scope/2  "sway"
  Ramp1/1 -> MATLAB System1/1
  Demux1/5 -> Scope1/5  "pitch"
  Demux1/2 -> Scope1/2  "sway"
  MATLAB System1/1 -> Demux1/1
  Mux/1 -> MATLAB Function/1(u)
  MATLAB System1/2 -> Terminator2/1
  MATLAB System/1 -> Demux/1
  MATLAB System/2 -> Terminator/1
  Demux/6 -> Mux/4, Scope/6  "yaw"
  Demux/5 -> Mux/3, Scope/5  "pitch"
  Demux1/4 -> Scope1/4  "roll"
  Demux1/3 -> Scope1/3  "heave"
  Ramp/1 -> MATLAB System/1

== system innerLoopForNav/innerLoop/HELI_CONT/UWV_CONT/Inner system/V_ned \ knots/Subsystem ==
  In3 : Inport
  MATLAB System1 : MATLABSystem  System=nedVelToBody  SimulateUsing=Code generation
      mask Type: nedVelToBody
      mask Display:
      | disp('nedVelToBody');
      | port_label('input',1,'V_ned');
      | port_label('input',2,'Euler');
      | port_label('output',1,'V_body');
  Mux : Mux  Inputs=2
  "trim : [phi, theta, psi]" : Selector  InputPortWidth=6  IndexOptions=Index vector (dialog)  Indices=[4 5 6]  OutputSizes=1
  "trim : [v_n, v_e, v_d]" : Selector  InputPortWidth=6  IndexOptions=Index vector (dialog)  Indices=[1 2 3]  OutputSizes=1
  trim_u,v,w,p,t,p : Outport
  wires:
  MATLAB System1/1 -> Mux/1  "trim_u,v,w"
  "trim : [phi, theta, psi]"/1 -> MATLAB System1/2, Mux/2  "trim_phi,theta,psi"
  "trim : [v_n, v_e, v_d]"/1 -> MATLAB System1/1
  Mux/1 -> trim_u,v,w,p,t,p/1, [trim]
  In3/1 -> "trim : [phi, theta, psi]"/1, "trim : [v_n, v_e, v_d]"/1

== matlab function innerLoopForNav/innerLoop/LAND_CMD/target_pos/PredictModel/MATLAB Function ==
  data: dy input; EI output; dz input; dphi input; dtheta input; ddy input; ddz input; phi input; theta input
function EI = EnergyIndex(dy, dz, dphi, dtheta, ddy, ddz, phi, theta)
% EI = 100 * dy * dy + 400 * ddy * ddy + dz * dz + ddz * ddz + 2500 * phi * phi + ...
%     2500 * dphi * dphi + theta * theta / 0.075 / 0.075 + 100 * dtheta * dtheta;
S = 1./[0.2, 2.0, 0.05, 0.2, 0.1, 2.0, 0.06, 0.15];
S = S.* S;
dstate = [dy, dz, dphi, dtheta, ddy, ddz, phi, theta];
EI = sum(S.*dstate.* dstate);

== matlab function innerLoopForNav/innerLoop/LAND_CMD/target_pos/PredictModel/ROA system/MATLAB Function ==
  data: u input; y output; isStop output
function [y, isStop] = fcn(u)

y = sqrt(u(1) * u(1) + u(2) * u(2) + u(3) * u(3) + u(4) * u(4));

if y > 0.15
    isStop = 0;
else
    isStop = 1;
end

== stateflow chart innerLoopForNav/innerLoop/LAND_CMD/target_pos/Chart ==
  state descent
    entry:
    target_pos = [-45;0;-13.4];
    state = 0;
    during:
    target_pos = [-45;0;-13.4];
    state = 0;
    exit:
    target_pos = [-45;0;-13.4];
    state = 0;
  state hover
    entry:
    target_pos = [-45;0;-13.4];
    state = 1;
    during:
    target_pos = [-45;0;-13.4];
    state = 1;
    exit:
    target_pos = [-45;0;-8.4];
    state = 1;
  state touchDown
    entry:
    target_pos = [-45;0;-8.4];
    state = 2;
    during:
    target_pos = [-45;0;-8.4];
    state = 2;
    exit:
    target_pos = [-45;0;-8.4];
    state = 2;
  (default) -> descent
  descent -> hover : [(z - target_pos(3)) * (z - target_pos(3)) + (x - target_pos(1) - ship_pos_x) * (x - target_pos(1) - ship_pos_x)<= 1e-1]
  hover -> touchDown : [EI <= 1.0]
  data: EI input; z input; target_pos output; state output; x input; ship_pos_x input

== matlab function innerLoopForNav/innerLoop/LAND_CMD/target_pos/Ship_motion/ROA system/MATLAB Function ==
  data: u input; y output; isStop output
function [y, isStop] = fcn(u)

y = sqrt(u(1) * u(1) + u(2) * u(2) + u(3) * u(3) + u(4) * u(4));

if y > 0.15
    isStop = 0;
else
    isStop = 1;
end

== matlab function innerLoopForNav/innerLoop/LAND_CMD/SCOPE_/MATLAB Function ==
  data: z input; shallStop output
function shallStop = fcn(z)
shallStop = 0;
if abs(z - 8.4) < 1e-2
    shallStop = 1;
end

== matlab function innerLoopForNav/innerLoop/LAND_CMD/target_pos/Ship_motion/MATLAB Function ==
  data: dy input; EI output; dz input; dphi input; dtheta input; ddy input; ddz input; phi input; theta input
function EI = EnergyIndex(dy, dz, dphi, dtheta, ddy, ddz, phi, theta)
% EI = 100 * dy * dy + 400 * ddy * ddy + dz * dz + ddz * ddz + 2500 * phi * phi + ...
%     2500 * dphi * dphi + theta * theta / 0.075 / 0.075 + 100 * dtheta * dtheta;
S = 1./[0.2, 2.0, 0.05, 0.2, 0.1, 2.0, 0.06, 0.15];
S = S.* S;
dstate = [dy, dz, dphi, dtheta, ddy, ddz, phi, theta];
EI = sum(S.*dstate.* dstate);
